simulink model "Stabilizer_QDrone_048378_OF"  (R2019a)
settings: Solver=ode2  StartTime=0.0  StopTime=inf  FixedStep=0.001  RelTol=1e-3  EnableMultiTasking=on
InitFcn:
  | addpath(fullfile(fileparts(get_param('Stabilizer_QDrone_048378_OF','FileName')),'optical_flow'));
model workspace (MAT data in the model file):
  MCOS : class17 (value not decoded)
  video_step_size = 0.06
undefined symbols (not defined in the file): datetime, gcbh, HIL, JPEG, m, OpticalFlow_, qc_get_step_size, QDrone_, saved_data, Stabilizer_, video_display_show
libraries: quarc_library x33, simulink_extras x5, simulink x4
(part 2 of 2)

== matlab function Stabilizer_QDrone_048378_OF/PHYSICAL PLANT w// LINEAR THRUST/Red - Low Voltage Green - Armed Blue - Disarmed/MATLAB Function LED Color Assignment ==
  data: arm input; value output; low_battery input
function value = fcn(arm, low_battery)

if low_battery
    value = 1;
elseif arm
    value = 2;
else 
    value = 3;
end
